simulink model "PV_BESS_EMS"  (R2026a)
settings: Solver=FixedStepDiscrete  StopTime=86400  FixedStep=900
undefined symbols (not defined in the file): E_batt_kWh, P_batt_max_kW, P_grid_limit_kW, precharge_enable
settings Model: Creator=陈进  LastModifiedBy=陈进

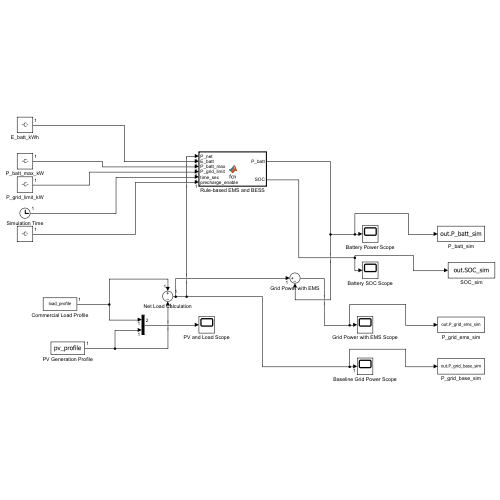
[thumbnail: Simulink's stored preview of the top-level diagram]
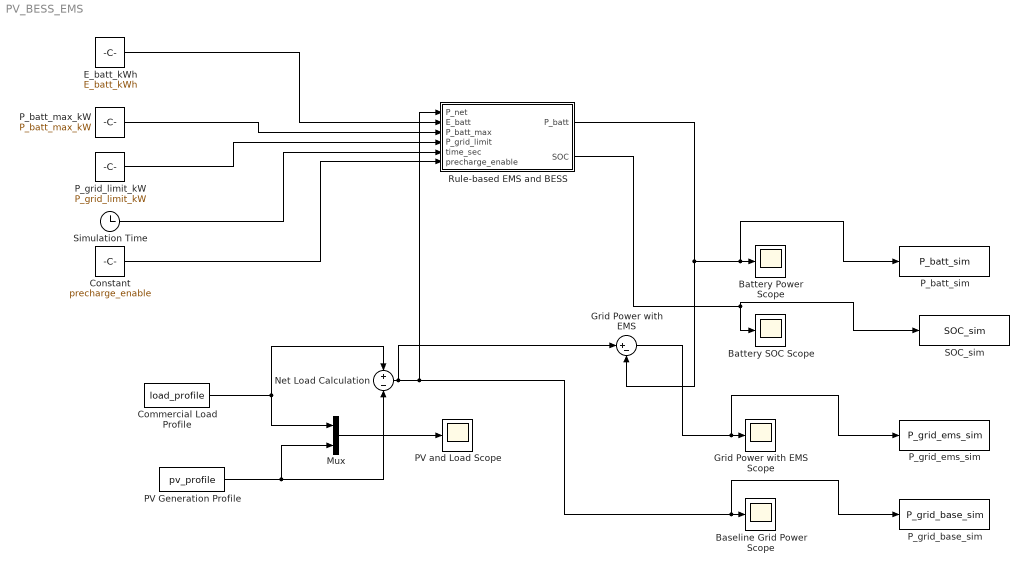
== system PV_BESS_EMS ==
  Baseline Grid Power Scope : Scope
      settings: ActiveDisplayYMinimum=-1  ActiveDisplayYMaximum=1
  Battery Power Scope : Scope
      settings: ActiveDisplayYMinimum=-1  ActiveDisplayYMaximum=1  DataLoggingVariableName=ScopeData4
  Battery SOC Scope : Scope
      settings: ActiveDisplayYMinimum=-1  ActiveDisplayYMaximum=1  DataLoggingVariableName=ScopeData3
  Commercial Load Profile : FromWorkspace  VariableName=load_profile
  Constant : Constant  Value=precharge_enable
  E_batt_kWh : Constant  Value=E_batt_kWh
  Grid Power with EMS : Sum  Inputs=|+-
  Grid Power with EMS Scope : Scope
      settings: ActiveDisplayYMinimum=-29.822290928643724  ActiveDisplayYMaximum=122.11599032135629  DataLoggingVariableName=ScopeData2
  Mux : Mux  Inputs=2
  Net Load Calculation : Sum  Inputs=+-
  PV Generation Profile : FromWorkspace  VariableName=pv_profile
  PV and Load Scope : Scope
      settings: ActiveDisplayYMinimum=-17.499999999999996  ActiveDisplayYMaximum=157.5
  P_batt_max_kW : Constant  Value=P_batt_max_kW
  P_batt_sim : ToWorkspace  VariableName=P_batt_sim  SaveFormat=Timeseries  SampleTime=-1
  P_grid_base_sim : ToWorkspace  VariableName=P_grid_base_sim  SaveFormat=Timeseries  SampleTime=-1
  P_grid_ems_sim : ToWorkspace  VariableName=P_grid_ems_sim  SaveFormat=Timeseries  SampleTime=-1
  P_grid_limit_kW : Constant  Value=P_grid_limit_kW
  Rule-based EMS and BESS : MATLAB Function  TreatAsAtomicUnit=on
  SOC_sim : ToWorkspace  VariableName=SOC_sim  SaveFormat=Timeseries  SampleTime=-1
  Simulation Time : Clock
  wires:
  Mux/1 -> PV and Load Scope/1
  Net Load Calculation/1 -> Grid Power with EMS/1, P_grid_base_sim/1, Baseline Grid Power Scope/1, Rule-based EMS and BESS/1(P_net)
  Commercial Load Profile/1 -> Mux/1, Net Load Calculation/1
  PV Generation Profile/1 -> Mux/2, Net Load Calculation/2
  Rule-based EMS and BESS/1(P_batt) -> Grid Power with EMS/2, P_batt_sim/1, Battery Power Scope/1
  Grid Power with EMS/1 -> P_grid_ems_sim/1, Grid Power with EMS Scope/1
  Rule-based EMS and BESS/2(SOC) -> Battery SOC Scope/1, SOC_sim/1
  E_batt_kWh/1 -> Rule-based EMS and BESS/2(E_batt)
  P_batt_max_kW/1 -> Rule-based EMS and BESS/3(P_batt_max)
  P_grid_limit_kW/1 -> Rule-based EMS and BESS/4(P_grid_limit)
  Simulation Time/1 -> Rule-based EMS and BESS/5(time_sec)
  Constant/1 -> Rule-based EMS and BESS/6(precharge_enable)

== matlab function PV_BESS_EMS/Rule-based EMS and BESS ==
  data: P_net input; P_batt output; SOC output; E_batt input; P_batt_max input; P_grid_limit input; time_sec input; precharge_enable input; SOC_initial parameter
function [P_batt, SOC] = fcn( ...
    P_net, E_batt, P_batt_max, P_grid_limit, ...
    time_sec, precharge_enable, SOC_initial)
% Rule-based EMS with forecast-based grid precharging
%
% P_net > 0: load demand exceeds PV generation
% P_net < 0: PV surplus is available
% P_batt > 0: battery discharging
% P_batt < 0: battery charging

%#codegen

%% Fixed simulation and battery parameters

dt = 900;                         % s, 15-minute interval

P_ch_max = P_batt_max;            % kW
P_dis_max = P_batt_max;           % kW

SOC_min = 0.20;
SOC_max = 0.90;

% Initial SOC is supplied by the simulation script
SOC_init = min(max(SOC_initial, SOC_min), SOC_max);

SOC_precharge_target = 0.90;

eta_ch = 0.95;
eta_dis = 0.95;

%% Battery state

persistent soc

if isempty(soc)
    soc = SOC_init;
end

%% Time information

% Single-day simulation: precharge only from 00:00 to before 06:00
% Excluding time_sec = 86400 prevents a false next-day charge step
is_precharge_window = ...
    (time_sec >= 0) && (time_sec < 6 * 3600);

%% EMS decision logic

% Default condition: battery idle
P_batt = 0;

% Rule 1: charge using PV surplus
if P_net < 0 && soc < SOC_max

    % Charging-power limit imposed by remaining SOC space
    P_charge_soc_max = ...
        (SOC_max - soc) * E_batt * 3600 ...
        / (eta_ch * dt);

    P_batt = -min( ...
        -P_net, ...
        min(P_ch_max, P_charge_soc_max));

% Rule 2: forecast-based off-peak grid precharging
elseif precharge_enable > 0.5 ...
        && is_precharge_window ...
        && soc < SOC_precharge_target ...
        && P_net < P_grid_limit

    % Charging power allowed by target SOC
    P_charge_soc_max = ...
        (SOC_precharge_target - soc) ...
        * E_batt * 3600 ...
        / (eta_ch * dt);

    % Available grid headroom before reaching grid limit
    P_grid_headroom = ...
        max(P_grid_limit - P_net, 0);

    % Grid charging uses only available headroom
    P_batt = -min( ...
        P_ch_max, ...
        min(P_charge_soc_max, P_grid_headroom));

% Rule 3: discharge for peak shaving
elseif P_net > P_grid_limit && soc > SOC_min

    % Discharging-power limit imposed by available SOC
    P_discharge_soc_max = ...
        (soc - SOC_min) * E_batt * 3600 ...
        * eta_dis / dt;

    P_batt = min( ...
        P_net - P_grid_limit, ...
        min(P_dis_max, P_discharge_soc_max));
end

%% SOC update

if P_batt < 0

    % Charging
    soc = soc + ...
        (-P_batt) * eta_ch * dt ...
        / (E_batt * 3600);

elseif P_batt > 0

    % Discharging
    soc = soc - ...
        P_batt * dt ...
        / (eta_dis * E_batt * 3600);
end

%% Numerical safety limits

soc = min(max(soc, SOC_min), SOC_max);

SOC = soc;
